simulink library "Linkage_Decoupled_DW"  (R2026a)
settings: Solver=VariableStepAuto
undefined symbols (not defined in the file): Ac, Af, Ar, InitLinkage, Left, Linkage, Visual, X, Y, Z
libraries: sm_lib x48, Suspension_Utilities x27, fl_lib x1, nesl_utility x1
(part 1 of 2)
Description:
  | Component of Simscape Vehicle Templates Library
  | 
  | Copyright 2018-2024 The MathWorks, Inc.
settings Model: Creator=smiller  LastModifiedBy=andrei

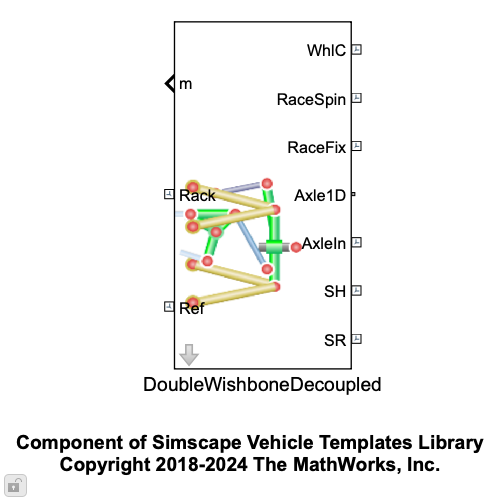
[thumbnail: Simulink's stored preview of the top-level diagram]
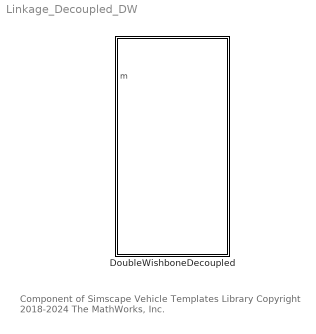
== system Linkage_Decoupled_DW ==
  note: Component of Simscape Vehicle Templates Library
      | Copyright 2018-2024 The MathWorks, Inc.
  DoubleWishboneDecoupled : Subsystem  VariantControl=DWDecoupled  mask(Double-Wishbone Suspension, Decoupled){popup_leftRight=Left, hp_in_f_ua=Linkage.UpperWishbone.sInboardF.Value, hp_in_r_ua=Linkage.UpperWishbone.sInboardR.Value, hp_out_ua=Linkage.UpperWishbone.sOutboard.Value, hp_in_f_la=Linkage.LowerWishbone.sInboardF.Value, hp_in_r_la=Linkage.LowerWishbone.sInboardR.Value, hp_out_la=Linkage.LowerWishbone.sOutboard.Value, hp_pushrod_in=Linkage.Pushrod.sBellcrank.Value, hp_pushrod_out=Linkage.Pushrod.sUpright.Value, hp_bcr_pivot=Linkage.Bellcrank.sPivot.Value, hp_bcr_shock_heaveL=Linkage.Shock.Heave.sLeft.Value, hp_bcr_shock_heaveR=Linkage.Shock.Heave.sRight.Value, hp_bcr_shock_rollL=Linkage.Shock.Roll.sLeft.Value, hp_bcr_shock_rollR=Linkage.Shock.Roll.sRight.Value, hp_upr_cg=Linkage.Upright.sCG.Value, hp_upr_wc=Linkage.Upright.sWheelCentre.Value, hp_in_rod=Linkage.TrackRod.sInboard.Value, hp_upr_rod=Linkage.TrackRod.sOutboard.Value, clr_hp=Visual.hp.clr, opc_hp=Visual.hp.opc, size_hp=Visual.hp.rad, Upper_Arm_to_Subframe=Linkage.Upper_Arm_to_Subframe, ua_mass=Linkage.UpperWishbone.m.Value, clr_ua=Visual.UpperArm.clr, opc_ua=Visual.part.opc, radius_ua=Visual.UpperArm.rad, Lower_Arm_to_Subframe=Linkage.Lower_Arm_to_Subframe, la_mass=Linkage.LowerWishbone.m.Value, clr_la=Visual.LowerArm.clr, opc_la=Visual.part.opc, radius_la=Visual.LowerArm.rad, upr_mass=Linkage.Upright.m.Value, atoe=Linkage.Upright.aToe.Value, acamber=Linkage.Upright.aCamber.Value, axle_len=Linkage.Upright.xAxle.Value, axle_whlc_to_bearing=Linkage.Upright.xWCtoBearing.Value, axle_mass=Linkage.Upright.mAxle.Value, clr_conn_upr=Visual.hp.clr, opc_conn_upr=Visual.hp.opc, size_conn_upr=Visual.hp.rad, clr_upr=Visual.Upright.clr, opc_upr=Visual.part.opc, radius_upr=Visual.Upright.rad, clr_axle=Visual.Axle.clr, opc_axle=Visual.part.opc, radius_axle=Visual.Axle.rad, rod_mass=Linkage.TrackRod.m.Value, clr_conn_rod=Visual.hp.clr, opc_conn_rod=Visual.hp.opc, size_conn_rod=Visual.hp.rad, clr_rod=Visual.TrackRod.clr, opc_rod=Visual.part.opc, radius_rod=Visual.TrackRod.rad, bcr_mass=Linkage.Bellcrank.m.Value, clr_bcr=Visual.Bellcrank.clr, opc_bcr=Visual.part.opc, radius_bcr=Visual.Bellcrank.rad, push_mass=Linkage.Pushrod.m.Value, clr_conn_push=Visual.hp.clr, opc_conn_push=Visual.hp.opc, size_conn_push=Visual.hp.rad, clr_push=Visual.Pushrod.clr, opc_push=Visual.part.opc, radius_push=Visual.Pushrod.rad, whl_init_spd_lr=InitLinkage.nWheel.Value}
      mask prompts: popup_leftRight "Left/Right"; hp_in_f_ua "Upper Arm Front [xyz] (m)"; hp_in_r_ua "Upper Arm Rear [xyz] (m)"; hp_out_ua "Upper Arm Outboard [xyz] (m)"; hp_in_f_la "Lower Arm Front [xyz] (m)"; hp_in_r_la "Lower Arm Rear [xyz] (m)"; hp_out_la "Lower Arm Outboard [xyz] (m)"; hp_pushrod_in "Pushrod Bellcrank [xyz] (m)"; hp_pushrod_out "Pushrod Upright [xyz] (m)"; hp_bcr_pivot "Bellcrank Pivot [xyz] (m)"; hp_bcr_shock_heaveL "Bellcrank Shock Heave Left [xyz] (m)"; hp_bcr_shock_heaveR "Bellcrank Shock Heave Right [xyz] (m)"; hp_bcr_shock_rollL "Bellcrank Shock Roll Left [xyz] (m)"; hp_bcr_shock_rollR "Bellcrank Shock Roll Right [xyz] (m)"; hp_upr_cg "Upright CG [xyz] (m)"; hp_upr_wc "Wheel Center [xyz] (m)"; hp_in_rod "Track Rod Inboard [xyz] (m)"; hp_upr_rod "Track Rod Outboard [xyz] (m)"; Upper_Arm_to_Subframe "Subframe Connection"; ua_mass "Mass (kg)"; clr_ua "Color [RGB]"; opc_ua "Opacity (0-1)"; radius_ua "Radius (m)"; Lower_Arm_to_Subframe "Subframe Connection"; la_mass "Mass (kg)"; clr_la "Color [RGB]"; opc_la "Opacity (0-1)"; radius_la "Radius (m)"; upr_mass "Mass (kg)"; atoe "Toe Angle (deg)"; acamber "Camber Angle (deg)"; axle_len "Axle Length (m)"; axle_whlc_to_bearing "Distance Wheel Ctr to Bearing (m)"; axle_mass "Axle Mass (kg)"; rod_mass "Mass (kg)"; bcr_mass "Mass (kg)"; push_mass "Mass (kg)"; whl_init_spd_lr "Initial Wheel Speed (rad/s)"
      mask help: This models a double-wishbone, decoupled suspension for steered configurations. Mechanical connections via a bellcrank permit this design to decouple stiffness and damping for body roll and heave.
      mask init:
      | if(popup_leftRight == 1)
      |     rhs_susp = 1;
      |     %whlind = 1;
      |     whl_init_spd = whl_init_spd_lr(1);
      |     hp_bcr_shock_heave = hp_bcr_shock_heaveL;
      |     hp_bcr_shock_roll = hp_bcr_shock_rollL;
      | elseif(popup_leftRight == 2)
      |     rhs_susp = -1;
      |     %whlind = 2;
      | 	whl_init_spd = whl_init_spd_lr(2);
      |     hp_bcr_shock_heave = hp_bcr_shock_heaveR;
      |     hp_bcr_shock_roll = hp_bcr_shock_rollR;
      | end
      mask Help: web('sm_car_doc_susp_double_wishbone.html')
      mask TypeOptions popup_leftRight: Hardpoints/popup_leftRight | Lower Arm/popup_leftRight | Upper Arm/popup_leftRight | Upright/popup_leftRight | Track Rod/popup_leftRight | Bellcrank/popup_leftRight | HP Bellcrank/popup_leftRight | Pushrod/popup_leftRight
      mask TypeOptions hp_in_f_ua: Upper Arm/hp_in_f | Hardpoints/hp_in_f_ua
      mask TypeOptions hp_in_r_ua: Upper Arm/hp_in_r | Hardpoints/hp_in_r_ua
      mask TypeOptions hp_out_ua: Upper Arm/hp_out | Upright/hp_ua_out
      mask TypeOptions hp_in_f_la: Hardpoints/hp_in_f_la | Lower Arm/hp_in_f
      mask TypeOptions hp_in_r_la: Hardpoints/hp_in_r_la | Lower Arm/hp_in_r
      mask TypeOptions hp_out_la: Upright/hp_la_out | Lower Arm/hp_out
      mask TypeOptions hp_pushrod_in: Pushrod/hp_in | Bellcrank/hp_pushrod | HP Bellcrank/hp_pushrod_in
      mask TypeOptions hp_pushrod_out: Pushrod/hp_out | Upright/hp_pushrod
      mask TypeOptions hp_bcr_pivot: Bellcrank/hp_bcr_pivot | HP Bellcrank/hp_bcr_pivot | Hardpoints/hp_bellcrank
      mask TypeOptions hp_upr_cg: Upright/hp_upr_cg
      mask TypeOptions hp_upr_wc: Upright/hp_upr_wc
      mask TypeOptions hp_in_rod: Track Rod/hp_in
      mask TypeOptions hp_upr_rod: Track Rod/hp_out | Upright/hp_upr_rod
      mask TypeOptions clr_hp: Hardpoints/clr_hp
      mask TypeOptions opc_hp: Hardpoints/opc_hp
      mask TypeOptions size_hp: Hardpoints/size_hp
      mask TypeOptions ua_mass: Upper Arm/ua_mass
      mask TypeOptions clr_ua: Upper Arm/clr_ua
      mask TypeOptions opc_ua: Upper Arm/opc_ua
      mask TypeOptions radius_ua: Upper Arm/radius_ua
      mask TypeOptions la_mass: Lower Arm/arm_mass
      mask TypeOptions clr_la: Lower Arm/clr_arm
      mask TypeOptions opc_la: Lower Arm/opc_arm
      mask TypeOptions radius_la: Lower Arm/radius_arm
      mask TypeOptions upr_mass: Upright/upr_mass
      mask TypeOptions atoe: Upright/atoe
      mask TypeOptions acamber: Upright/acamber
      mask TypeOptions axle_len: Upright/axle_len
      mask TypeOptions axle_whlc_to_bearing: Upright/axle_whlc_to_bearing
      mask TypeOptions axle_mass: Upright/axle_mass
      mask TypeOptions clr_conn_upr: Upright/clr_conn_upr
      mask TypeOptions opc_conn_upr: Upright/opc_conn_upr
      mask TypeOptions size_conn_upr: Upright/size_conn_upr
      mask TypeOptions clr_upr: Upright/clr_upr
      mask TypeOptions opc_upr: Upright/opc_upr
      mask TypeOptions radius_upr: Upright/radius_upr
      mask TypeOptions clr_axle: Upright/clr_axle
      mask TypeOptions opc_axle: Upright/opc_axle
      mask TypeOptions radius_axle: Upright/radius_axle
      mask TypeOptions rod_mass: Track Rod/rod_mass
      mask TypeOptions clr_conn_rod: Track Rod/clr_conn_rod
      mask TypeOptions opc_conn_rod: Track Rod/opc_conn_rod
      mask TypeOptions size_conn_rod: Track Rod/size_conn_rod
      mask TypeOptions clr_rod: Track Rod/clr_rod
      mask TypeOptions opc_rod: Track Rod/opc_rod
      mask TypeOptions radius_rod: Track Rod/radius_rod
      mask TypeOptions bcr_mass: Bellcrank/bcr_mass
      mask TypeOptions clr_bcr: Bellcrank/clr_bcr
      mask TypeOptions opc_bcr: Bellcrank/opc_bcr
      mask TypeOptions radius_bcr: Bellcrank/radius_bcr
      mask TypeOptions push_mass: Pushrod/rod_mass
      mask TypeOptions clr_conn_push: Pushrod/clr_conn_rod
      mask TypeOptions opc_conn_push: Pushrod/opc_conn_rod
      mask TypeOptions size_conn_push: Pushrod/size_conn_rod
      mask TypeOptions clr_push: Pushrod/clr_rod
      mask TypeOptions opc_push: Pushrod/opc_rod
      mask TypeOptions radius_push: Pushrod/radius_rod
      mask DialogControl cont_hp Prompt: Hardpoints
      mask DialogControl cont_vis_hp Prompt: Visualization
      mask DialogControl text_clr_hp Prompt: Color [RGB]
      mask DialogControl text_opc_hp Prompt: Opac. (0-1)
      mask DialogControl text_size_hp Prompt: Size (m)
      mask DialogControl text_hp Prompt: Hardpoints
      mask DialogControl cont_ua Prompt: UA
      mask DialogControl cont_vis_ua Prompt: Visualization
      mask DialogControl cont_la Prompt: LA
      mask DialogControl cont_vis_la Prompt: Visualization
      mask DialogControl cont_upright Prompt: Upright
      mask DialogControl grp_upright Prompt: Upright
      mask DialogControl grp_upright_axle Prompt: Axle
      mask DialogControl cont_vis_upr Prompt: Visualization
      mask DialogControl text_clr_upr Prompt: Color [RGB]
      mask DialogControl text_opc_upr Prompt: Opac. (0-1)
      mask DialogControl text_size_upr Prompt: Size (m)
      mask DialogControl text_conn_upr Prompt: Connections
      mask DialogControl text_upright Prompt: Upright
      mask DialogControl text_axle Prompt: Axle
      mask DialogControl cont_steer Prompt: Steer
      mask DialogControl grp_rod Prompt: Rod
      mask DialogControl cont_vis_rod Prompt: Visualization
      mask DialogControl text_clr_rod Prompt: Color [RGB]
      mask DialogControl text_opc_rod Prompt: Opac. (0-1)
      mask DialogControl text_size_rod Prompt: Size (m)
      mask DialogControl text_conn_rod Prompt: Connections
      mask DialogControl text_rod_rod Prompt: Rod
      mask DialogControl cont_bellcrank Prompt: Bellcrank
      mask DialogControl grp_bellcrank Prompt: Bellcrank
      mask DialogControl cont_vis_bellcrank Prompt: Visualization
      mask DialogControl text_clr_bellcrank Prompt: Color [RGB]
      mask DialogControl text_opc_bellcrank Prompt: Opac. (0-1)
      mask DialogControl text_size_bellcrank Prompt: Size (m)
      mask DialogControl text_bellcrank Prompt: Bellcrank
      mask DialogControl cont_push Prompt: Pushrod
      mask DialogControl cont_vis_pushrod Prompt: Visualization
      mask DialogControl text_clr_push Prompt: Color [RGB]
      mask DialogControl text_opc_push Prompt: Opac. (0-1)
      mask DialogControl text_size_push Prompt: Size (m)
      mask DialogControl text_push Prompt: Connections
      mask DialogControl text_rod Prompt: Rod
      mask DialogControl cont_init Prompt: Initial
      mask Display: image('sm_car_vehicle_linkage_dwdec_IMAGE.png');

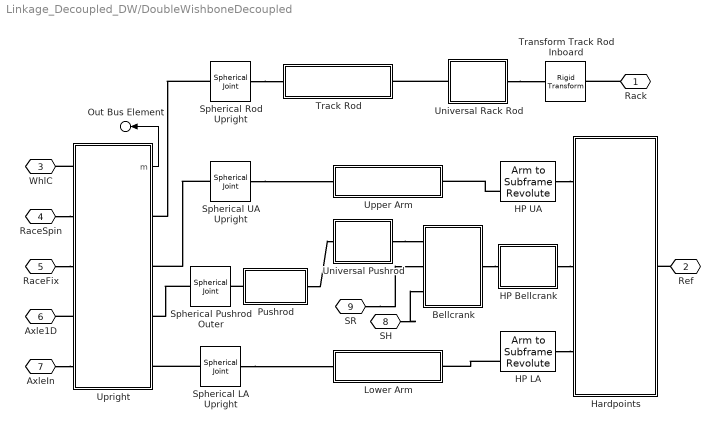
== system Linkage_Decoupled_DW/DoubleWishboneDecoupled ==
  Bellcrank : Subsystem  mask(Bellcrank){popup_leftRight=Left, hp_bcr_pivot=hp_bcr_pivot, hp_bcr_shock_heave=hp_bcr_shock_heave, hp_bcr_shock_roll=hp_bcr_shock_roll, hp_pushrod=hp_pushrod_in, bcr_mass=bcr_mass, clr_bcr=clr_bcr, opc_bcr=opc_bcr, radius_bcr=radius_bcr}
      mask prompts: popup_leftRight "Left/Right"; hp_bcr_pivot "HP Bellcrank Pivot [xyz] (m)"; hp_bcr_shock_heave "HP Bellcrank Shock Heave [xyz] (m)"; hp_bcr_shock_roll "HP Bellcrank Shock Roll [xyz] (m)"; hp_pushrod "HP Bellcrank Pushrod [xyz] (m)"; bcr_mass "Mass (kg)"; clr_bcr "Color [RGB]"; opc_bcr "Opacity (0-1)"; radius_bcr "Radius (m)"
      mask help: Models a bellcrank with one pivot and 3 attachment points. The axis of the pivot is normal to the plane formed by the pivot, connection to the pushrod, and connection to the shock.
      mask init:
      | if(popup_leftRight == 1)
      |     rhs_susp = 1;
      |     %hp_shock_roll = hp_bcr_shock_roll; % Use left value
      | elseif(popup_leftRight == 2)
      |     rhs_susp = -1;
      |     % Code to mirror hardpoint about vehicle xz plane 
      |     % and the plane defined by the bellcrank pivot axis
      |     % and the y axis of the vehicle
      |     % Code not used so that points can be specified independently
      |     % Left here as a reference.
      |     %{
      |     a1 = atan2(hp_pushrod(1)-hp_bcr_pivot(1)   ,hp_pushrod(3)-hp_bcr_pivot(3));
      |     a2 = atan2(hp_bcr_shock_roll(1)-hp_bcr_pivot(1),hp_bcr_shock_roll(3)-hp_bcr_pivot(3));
      |     d_roll2piv = norm(hp_bcr_shock_roll([1 3])-hp_bcr_pivot([1 3]));
      |     d_roll_mirror_axis = d_roll2piv*cos(a2-a1);
      |     mirr_dx = d_roll_mirror_axis*sin(a1);
      |     mirr_dz = d_roll_mirror_axis*cos(a1);
      |     hp_shock_roll = ...
      |         [hp_bcr_shock_roll(1)-2*mirr_dx -hp_bcr_shock_roll(2) hp_bcr_shock_roll(3)-2*mirr_dz];
      |     %}
      | end
      | 
      | rhs_hp = [1 rhs_susp 1];
      mask TypeOptions popup_leftRight: Left | Right
      mask TypeOptions clr_bcr: Arm Pivot Shock Roll/clr_solid | Arm Pivot Push/clr_solid | Arm Pivot Shock Heave/clr_solid | Arm Push Shock/clr_solid
      mask TypeOptions opc_bcr: Arm Pivot Shock Roll/opc_solid | Arm Pivot Push/opc_solid | Arm Pivot Shock Heave/opc_solid | Arm Push Shock/opc_solid
      mask TypeOptions radius_bcr: Arm Pivot Shock Roll/rad_solid | Arm Pivot Push/rad_solid | Arm Pivot Shock Heave/rad_solid | Arm Push Shock/rad_solid
      mask DialogControl cont_ua Prompt: UA
      mask DialogControl cont_vis_ua Prompt: Visualization
      mask Display: image('sm_car_vehicle_linkage_bellcrank_IMAGE.png');
  HP Bellcrank : Subsystem  mask(Revolute Joint 3 Points){popup_leftRight=Left, hp_bcr_pivot=hp_bcr_pivot, hp_pushrod_in=hp_pushrod_in, hp_bcr_shock=hp_bcr_shock_heave}
      mask prompts: popup_leftRight "Left/Right"; hp_bcr_pivot "HP Bellcrank Pivot [xyz] (m)"; hp_pushrod_in "HP Pushrod Inner [xyz] (m)"; hp_bcr_shock "HP Bellcrank Shock Heave [xyz] (m)"
      mask help: Revolute Joint with degree of freedom normal to 3 hardpoints.
      mask init:
      | % Set parameter for mirroring (+y or -y)
      | if(popup_leftRight == 1)
      |     rhs_susp = 1;    
      | elseif(popup_leftRight == 2)
      |     rhs_susp = -1;
      | end
      | 
      | rhs_hp = [1 rhs_susp 1];
      mask TypeOptions popup_leftRight: Left | Right
      mask Display: image('sm_car_variant_revolute.png')
  HP LA : Suspension_Utilities/Arm to Subframe Revolute  VariantControl=Variant1  LabelModeActiveChoice=Bushing_AxRad  popup_leftRight=Left  hp_f=hp_in_f_ua  hp_r=hp_in_r_ua  Connection=Lower_Arm_to_Subframe  VariantLabel=Lower_Arm_to_Subframe.class.Value
      settings: AttributesFormatString=%<ActiveVariant>  SourceProductName=SmCar - Suspension Utilites
  HP UA : Suspension_Utilities/Arm to Subframe Revolute  VariantControl=Variant1  LabelModeActiveChoice=Bushing_AxRad  popup_leftRight=Left  hp_f=hp_in_f_ua  hp_r=hp_in_r_ua  Connection=Upper_Arm_to_Subframe  VariantLabel=Upper_Arm_to_Subframe.class.Value
      settings: AttributesFormatString=%<ActiveVariant>  SourceProductName=SmCar - Suspension Utilites
  Hardpoints : Subsystem  mask{popup_leftRight=Left, hp_in_f_ua=hp_in_f_ua, hp_in_r_ua=hp_in_r_ua, hp_in_f_la=hp_in_f_la, hp_in_r_la=hp_in_r_la, hp_bellcrank=hp_bcr_pivot, clr_hp=clr_hp, opc_hp=opc_hp, size_hp=size_hp}
      mask prompts: popup_leftRight "Left/Right"; hp_in_f_ua "Upper Arm Front [xyz] (m)"; hp_in_r_ua "Upper Arm Rear [xyz] (m)"; hp_in_f_la "Lower Arm Front [xyz] (m)"; hp_in_r_la "Lower Arm Rear [xyz] (m)"; hp_bellcrank "Bellcrank Pivot [xyz] (m)"
      mask init:
      | % Set parameter for mirroring (+y or -y)
      | if(popup_leftRight == 1)
      |     rhs_susp = 1;    
      | elseif(popup_leftRight == 2)
      |     rhs_susp = -1;
      | end
      | 
      | rhs_hp = [1 rhs_susp 1];
      mask TypeOptions popup_leftRight: Left | Right
      mask TypeOptions clr_hp: Subsystem/Vis HP LAf/GraphicDiffuseColor | Vis HP LAr/GraphicDiffuseColor | Vis HP Bellcrank/GraphicDiffuseColor | Vis HP UAf/GraphicDiffuseColor | Vis HP UAr/GraphicDiffuseColor
      mask TypeOptions opc_hp: Subsystem/Vis HP LAf/GraphicOpacity | Vis HP LAr/GraphicOpacity | Vis HP Bellcrank/GraphicOpacity | Vis HP UAf/GraphicOpacity | Vis HP UAr/GraphicOpacity
      mask DialogControl cont_hp Prompt: Hardpoints
      mask DialogControl cont_vis_hp Prompt: Visualization
      mask DialogControl text_clr_hp Prompt: Color [RGB]
      mask DialogControl text_opc_hp Prompt: Opac. (0-1)
      mask DialogControl text_size_hp Prompt: Size (m)
      mask DialogControl text_hp Prompt: Hardpoints
      mask Display: image('sm_car_vehicle_linkage_dw_hp_IMAGE.png');
  Lower Arm : Subsystem  mask{popup_leftRight=Left, hp_in_f=hp_in_f_la, hp_in_r=hp_in_r_la, hp_out=hp_out_la, arm_mass=la_mass, clr_arm=clr_la, opc_arm=opc_la, radius_arm=radius_la}
      mask prompts: popup_leftRight "Left/Right"; hp_in_f "Inboard Front [xyz] (m)"; hp_in_r "Inboard Rear [xyz] (m)"; hp_out "Outboard [xyz] (m)"; arm_mass "Mass (kg)"; clr_arm "Color [RGB]"; opc_arm "Opacity (0-1)"; radius_arm "Radius (m)"
      mask init:
      | if(popup_leftRight == 1)
      |     rhs_susp = 1;
      | elseif(popup_leftRight == 2)
      |     rhs_susp = -1;
      | end
      | 
      | rhs_hp = [1 rhs_susp 1];
      mask TypeOptions popup_leftRight: Left | Right
      mask TypeOptions clr_arm: Arm F/clr_solid | Arm R/clr_solid
      mask TypeOptions opc_arm: Arm F/opc_solid | Arm R/opc_solid
      mask TypeOptions radius_arm: Arm F/rad_solid | Arm R/rad_solid
      mask DialogControl cont_ua Prompt: LA
      mask DialogControl cont_vis_arm Prompt: Visualization
      mask Display: image('sm_car_vehicle_linkage_dw_ua_IMAGE.png');
  Pushrod : Subsystem  VariantControl=Steer  mask{popup_leftRight=Left, hp_in=hp_pushrod_in, hp_out=hp_pushrod_out, rod_mass=push_mass, clr_conn_rod=clr_conn_push, opc_conn_rod=opc_conn_push, size_conn_rod=size_conn_push, clr_rod=clr_push, opc_rod=opc_push, radius_rod=radius_push}
      mask prompts: popup_leftRight "Left/Right"; hp_in "Inboard [xyz] (m)"; hp_out "Outboard [xyz] (m)"; rod_mass "Mass (kg)"
      mask init:
      | if(popup_leftRight == 1)
      |     rhs_rod = 1;
      | elseif(popup_leftRight == 2)
      |     rhs_rod = -1;
      | end
      mask TypeOptions popup_leftRight: Left | Right
      mask TypeOptions rod_mass: Arm/Mass
      mask TypeOptions clr_conn_rod:
      | Vis
      | Upright
      | Steer/GraphicDiffuseColor | Vis
      | Rack
      | Rod/GraphicDiffuseColor
      mask TypeOptions opc_conn_rod:
      | Vis
      | Upright
      | Steer/GraphicOpacity | Vis
      | Rack
      | Rod/GraphicOpacity
      mask TypeOptions clr_rod: Arm/clr_solid
      mask TypeOptions opc_rod: Arm/opc_solid
      mask TypeOptions radius_rod: Arm/rad_solid
      mask DialogControl cont_rod Prompt: Rod
      mask DialogControl grp_rod Prompt: Rod
      mask DialogControl cont_vis_rod Prompt: Visualization
      mask DialogControl text_clr_rod Prompt: Color [RGB]
      mask DialogControl text_opc_rod Prompt: Opacity (0-1)
      mask DialogControl text_size_rod Prompt: Radius (m)
      mask DialogControl text_conn_rod Prompt: Connections
      mask DialogControl text_rod_rod Prompt: Rod
      mask Display: image('sm_car_vehicle_linkage_link_IMAGE.png');
  Spherical LA Upright : sm_lib/Joints/Spherical Joint  JointMode=Normal  CompositeWrenchDir=FollowerOnBase  CompositeWrenchFrame=BaseFrame  SenseConstraintForce=off  SenseConstraintTorque=off  SenseTotalForce=off  SenseTotalTorque=off  PositionTargetSpecify=off  PositionTargetPriority=High  PositionTargetRotationMethod=None  PositionTargetFollAlignAxisA=+X  PositionTargetBaseAlignAxisA=+Y  PositionTargetFollAlignAxisB=+Y  PositionTargetBaseAlignAxisB=+Z  PositionTargetRotationStandardAxis=+Z  PositionTargetRotationAngle=0.0  PositionTargetRotationAngleUnits=deg  PositionTargetRotationArbitraryAxis=[0 0 1]  PositionTargetRotationSequenceAxes=FollowerAxes  PositionTargetRotationSequence=XYX  PositionTargetRotationSequenceAngles=[0 0 0]  PositionTargetRotationSequenceAnglesUnits=deg  PositionTargetRotationMatrix=[1 0 0; 0 1 0; 0 0 1]  PositionTargetQuaternion=[1 0 0 0]  VelocityTargetSpecify=off  VelocityTargetPriority=High  VelocityTargetValue=[0 0 0]  VelocityTargetValueUnits=deg/s  VelocityTargetInFollowerFrame=on  EqPosRotationMethod=None  EqPosFollAlignAxisA=+X  EqPosBaseAlignAxisA=+Y  EqPosFollAlignAxisB=+Y  EqPosBaseAlignAxisB=+Z  EqPosRotationStandardAxis=+Z  EqPosRotationAngle=0.0  EqPosRotationAngleUnits=deg  EqPosRotationArbitraryAxis=[0 0 1]  EqPosRotationSequenceAxes=FollowerAxes  EqPosRotationSequence=XYX  EqPosRotationSequenceAngles=[0 0 0]  EqPosRotationSequenceAnglesUnits=deg  EqPosRotationMatrix=[1 0 0; 0 1 0; 0 0 1]  EqPosQuaternion=[1 0 0 0]  SpringStiffness=0  SpringStiffnessUnits=N*m/deg  DampingCoefficient=0  DampingCoefficientUnits=N*m/(deg/s)  LowerLimitSpecify=off  LowerLimitBound=15  LowerLimitBoundUnits=deg  LowerLimitStiffness=1e4  LowerLimitStiffnessUnits=N*m/deg  LowerLimitDamping=10  LowerLimitDampingUnits=N*m/(deg/s)  LowerLimitTransitionRegionWidth=0.1  LowerLimitTransitionRegionWidthUnits=deg  UpperLimitSpecify=off  UpperLimitBound=45  UpperLimitBoundUnits=deg  UpperLimitStiffness=1e4  UpperLimitStiffnessUnits=N*m/deg  UpperLimitDamping=10  UpperLimitDampingUnits=N*m/(deg/s)  UpperLimitTransitionRegionWidth=0.1  UpperLimitTransitionRegionWidthUnits=deg  TorqueActuationMode=NoTorque  ActuateTorqueX=off  ActuateTorqueY=off  ActuateTorqueZ=off  ActuateTorque=off  ActuationFrame=BaseFrame  SensePosition=off  SenseVelocityX=off  SenseVelocityY=off  SenseVelocityZ=off  SenseVelocity=off  SenseAccelerationX=off  SenseAccelerationY=off  SenseAccelerationZ=off  SenseAcceleration=off  SenseLowerLimitTorqueMag=off  SenseUpperLimitTorqueMag=off  SensingFrame=BaseFrame
  Spherical Pushrod Outer : sm_lib/Joints/Spherical Joint  JointMode=Normal  CompositeWrenchDir=FollowerOnBase  CompositeWrenchFrame=BaseFrame  SenseConstraintForce=off  SenseConstraintTorque=off  SenseTotalForce=off  SenseTotalTorque=off  PositionTargetSpecify=on  PositionTargetPriority=Low  PositionTargetRotationMethod=AlignedAxes  PositionTargetFollAlignAxisA=+X  PositionTargetBaseAlignAxisA=+X  PositionTargetFollAlignAxisB=+Y  PositionTargetBaseAlignAxisB=+Y  PositionTargetRotationStandardAxis=+Z  PositionTargetRotationAngle=0.0  PositionTargetRotationAngleUnits=deg  PositionTargetRotationArbitraryAxis=[0 0 1]  PositionTargetRotationSequenceAxes=FollowerAxes  PositionTargetRotationSequence=XYX  PositionTargetRotationSequenceAngles=[0 0 0]  PositionTargetRotationSequenceAnglesUnits=deg  PositionTargetRotationMatrix=[1 0 0; 0 1 0; 0 0 1]  PositionTargetQuaternion=[1 0 0 0]  VelocityTargetSpecify=off  VelocityTargetPriority=High  VelocityTargetValue=[0 0 0]  VelocityTargetValueUnits=deg/s  VelocityTargetInFollowerFrame=on  EqPosRotationMethod=None  EqPosFollAlignAxisA=+X  EqPosBaseAlignAxisA=+Y  EqPosFollAlignAxisB=+Y  EqPosBaseAlignAxisB=+Z  EqPosRotationStandardAxis=+Z  EqPosRotationAngle=0.0  EqPosRotationAngleUnits=deg  EqPosRotationArbitraryAxis=[0 0 1]  EqPosRotationSequenceAxes=FollowerAxes  EqPosRotationSequence=XYX  EqPosRotationSequenceAngles=[0 0 0]  EqPosRotationSequenceAnglesUnits=deg  EqPosRotationMatrix=[1 0 0; 0 1 0; 0 0 1]  EqPosQuaternion=[1 0 0 0]  SpringStiffness=0  SpringStiffnessUnits=N*m/deg  DampingCoefficient=0  DampingCoefficientUnits=N*m/(deg/s)  LowerLimitSpecify=off  LowerLimitBound=15  LowerLimitBoundUnits=deg  LowerLimitStiffness=1e4  LowerLimitStiffnessUnits=N*m/deg  LowerLimitDamping=10  LowerLimitDampingUnits=N*m/(deg/s)  LowerLimitTransitionRegionWidth=0.1  LowerLimitTransitionRegionWidthUnits=deg  UpperLimitSpecify=off  UpperLimitBound=45  UpperLimitBoundUnits=deg  UpperLimitStiffness=1e4  UpperLimitStiffnessUnits=N*m/deg  UpperLimitDamping=10  UpperLimitDampingUnits=N*m/(deg/s)  UpperLimitTransitionRegionWidth=0.1  UpperLimitTransitionRegionWidthUnits=deg  TorqueActuationMode=NoTorque  ActuateTorqueX=off  ActuateTorqueY=off  ActuateTorqueZ=off  ActuateTorque=off  ActuationFrame=BaseFrame  SensePosition=off  SenseVelocityX=off  SenseVelocityY=off  SenseVelocityZ=off  SenseVelocity=off  SenseAccelerationX=off  SenseAccelerationY=off  SenseAccelerationZ=off  SenseAcceleration=off  SenseLowerLimitTorqueMag=off  SenseUpperLimitTorqueMag=off  SensingFrame=BaseFrame
  Spherical Rod Upright : sm_lib/Joints/Spherical Joint  JointMode=Normal  CompositeWrenchDir=FollowerOnBase  CompositeWrenchFrame=BaseFrame  SenseConstraintForce=off  SenseConstraintTorque=off  SenseTotalForce=off  SenseTotalTorque=off  PositionTargetSpecify=off  PositionTargetPriority=High  PositionTargetRotationMethod=None  PositionTargetFollAlignAxisA=+X  PositionTargetBaseAlignAxisA=+Y  PositionTargetFollAlignAxisB=+Y  PositionTargetBaseAlignAxisB=+Z  PositionTargetRotationStandardAxis=+Z  PositionTargetRotationAngle=0.0  PositionTargetRotationAngleUnits=deg  PositionTargetRotationArbitraryAxis=[0 0 1]  PositionTargetRotationSequenceAxes=FollowerAxes  PositionTargetRotationSequence=XYX  PositionTargetRotationSequenceAngles=[0 0 0]  PositionTargetRotationSequenceAnglesUnits=deg  PositionTargetRotationMatrix=[1 0 0; 0 1 0; 0 0 1]  PositionTargetQuaternion=[1 0 0 0]  VelocityTargetSpecify=off  VelocityTargetPriority=High  VelocityTargetValue=[0 0 0]  VelocityTargetValueUnits=deg/s  VelocityTargetInFollowerFrame=on  EqPosRotationMethod=None  EqPosFollAlignAxisA=+X  EqPosBaseAlignAxisA=+Y  EqPosFollAlignAxisB=+Y  EqPosBaseAlignAxisB=+Z  EqPosRotationStandardAxis=+Z  EqPosRotationAngle=0.0  EqPosRotationAngleUnits=deg  EqPosRotationArbitraryAxis=[0 0 1]  EqPosRotationSequenceAxes=FollowerAxes  EqPosRotationSequence=XYX  EqPosRotationSequenceAngles=[0 0 0]  EqPosRotationSequenceAnglesUnits=deg  EqPosRotationMatrix=[1 0 0; 0 1 0; 0 0 1]  EqPosQuaternion=[1 0 0 0]  SpringStiffness=0  SpringStiffnessUnits=N*m/deg  DampingCoefficient=0  DampingCoefficientUnits=N*m/(deg/s)  LowerLimitSpecify=off  LowerLimitBound=15  LowerLimitBoundUnits=deg  LowerLimitStiffness=1e4  LowerLimitStiffnessUnits=N*m/deg  LowerLimitDamping=10  LowerLimitDampingUnits=N*m/(deg/s)  LowerLimitTransitionRegionWidth=0.1  LowerLimitTransitionRegionWidthUnits=deg  UpperLimitSpecify=off  UpperLimitBound=45  UpperLimitBoundUnits=deg  UpperLimitStiffness=1e4  UpperLimitStiffnessUnits=N*m/deg  UpperLimitDamping=10  UpperLimitDampingUnits=N*m/(deg/s)  UpperLimitTransitionRegionWidth=0.1  UpperLimitTransitionRegionWidthUnits=deg  TorqueActuationMode=NoTorque  ActuateTorqueX=off  ActuateTorqueY=off  ActuateTorqueZ=off  ActuateTorque=off  ActuationFrame=BaseFrame  SensePosition=off  SenseVelocityX=off  SenseVelocityY=off  SenseVelocityZ=off  SenseVelocity=off  SenseAccelerationX=off  SenseAccelerationY=off  SenseAccelerationZ=off  SenseAcceleration=off  SenseLowerLimitTorqueMag=off  SenseUpperLimitTorqueMag=off  SensingFrame=BaseFrame
  Spherical UA Upright : sm_lib/Joints/Spherical Joint  JointMode=Normal  CompositeWrenchDir=FollowerOnBase  CompositeWrenchFrame=BaseFrame  SenseConstraintForce=off  SenseConstraintTorque=off  SenseTotalForce=off  SenseTotalTorque=off  PositionTargetSpecify=on  PositionTargetPriority=High  PositionTargetRotationMethod=StandardAxis  PositionTargetFollAlignAxisA=+X  PositionTargetBaseAlignAxisA=+Y  PositionTargetFollAlignAxisB=+Y  PositionTargetBaseAlignAxisB=+Z  PositionTargetRotationStandardAxis=+Z  PositionTargetRotationAngle=0.0  PositionTargetRotationAngleUnits=deg  PositionTargetRotationArbitraryAxis=[0 0 1]  PositionTargetRotationSequenceAxes=FollowerAxes  PositionTargetRotationSequence=XYX  PositionTargetRotationSequenceAngles=[0 0 0]  PositionTargetRotationSequenceAnglesUnits=deg  PositionTargetRotationMatrix=[1 0 0; 0 1 0; 0 0 1]  PositionTargetQuaternion=[1 0 0 0]  VelocityTargetSpecify=off  VelocityTargetPriority=High  VelocityTargetValue=[0 0 0]  VelocityTargetValueUnits=deg/s  VelocityTargetInFollowerFrame=on  EqPosRotationMethod=None  EqPosFollAlignAxisA=+X  EqPosBaseAlignAxisA=+Y  EqPosFollAlignAxisB=+Y  EqPosBaseAlignAxisB=+Z  EqPosRotationStandardAxis=+Z  EqPosRotationAngle=0.0  EqPosRotationAngleUnits=deg  EqPosRotationArbitraryAxis=[0 0 1]  EqPosRotationSequenceAxes=FollowerAxes  EqPosRotationSequence=XYX  EqPosRotationSequenceAngles=[0 0 0]  EqPosRotationSequenceAnglesUnits=deg  EqPosRotationMatrix=[1 0 0; 0 1 0; 0 0 1]  EqPosQuaternion=[1 0 0 0]  SpringStiffness=0  SpringStiffnessUnits=N*m/deg  DampingCoefficient=0  DampingCoefficientUnits=N*m/(deg/s)  LowerLimitSpecify=off  LowerLimitBound=15  LowerLimitBoundUnits=deg  LowerLimitStiffness=1e4  LowerLimitStiffnessUnits=N*m/deg  LowerLimitDamping=10  LowerLimitDampingUnits=N*m/(deg/s)  LowerLimitTransitionRegionWidth=0.1  LowerLimitTransitionRegionWidthUnits=deg  UpperLimitSpecify=off  UpperLimitBound=45  UpperLimitBoundUnits=deg  UpperLimitStiffness=1e4  UpperLimitStiffnessUnits=N*m/deg  UpperLimitDamping=10  UpperLimitDampingUnits=N*m/(deg/s)  UpperLimitTransitionRegionWidth=0.1  UpperLimitTransitionRegionWidthUnits=deg  TorqueActuationMode=NoTorque  ActuateTorqueX=off  ActuateTorqueY=off  ActuateTorqueZ=off  ActuateTorque=off  ActuationFrame=BaseFrame  SensePosition=off  SenseVelocityX=off  SenseVelocityY=off  SenseVelocityZ=off  SenseVelocity=off  SenseAccelerationX=off  SenseAccelerationY=off  SenseAccelerationZ=off  SenseAcceleration=off  SenseLowerLimitTorqueMag=off  SenseUpperLimitTorqueMag=off  SensingFrame=BaseFrame
  Track Rod : Subsystem  VariantControl=Steer  mask{popup_leftRight=Left, hp_in=hp_in_rod, hp_out=hp_upr_rod, rod_mass=rod_mass, clr_conn_rod=clr_conn_rod, opc_conn_rod=opc_conn_rod, size_conn_rod=size_conn_rod, clr_rod=clr_rod, opc_rod=opc_rod, radius_rod=radius_rod}
      mask prompts: popup_leftRight "Left/Right"; hp_in "Inboard [xyz] (m)"; hp_out "Outboard [xyz] (m)"; rod_mass "Mass (kg)"; clr_rod "Color [RGB]"; opc_rod "Opacity (0-1)"; radius_rod "Radius (m)"
      mask init:
      | if(popup_leftRight == 1)
      |     rhs_rod = 1;
      | elseif(popup_leftRight == 2)
      |     rhs_rod = -1;
      | end
      mask TypeOptions popup_leftRight: Left | Right
      mask TypeOptions rod_mass: Rod/Mass
      mask TypeOptions clr_conn_rod:
      | Vis
      | Upright
      | Steer/GraphicDiffuseColor | Vis
      | Rack
      | Rod/GraphicDiffuseColor
      mask TypeOptions opc_conn_rod:
      | Vis
      | Upright
      | Steer/GraphicOpacity | Vis
      | Rack
      | Rod/GraphicOpacity
      mask TypeOptions clr_rod: Rod/clr_solid
      mask TypeOptions opc_rod: Rod/opc_solid
      mask TypeOptions radius_rod: Rod/rad_solid
      mask DialogControl cont_rod Prompt: Rod
      mask DialogControl grp_rod Prompt: Rod
      mask DialogControl cont_vis_rod Prompt: Visualization
      mask DialogControl text_clr_rod Prompt: Color [RGB]
      mask DialogControl text_opc_rod Prompt: Opac. (0-1)
      mask DialogControl text_size_rod Prompt: Size (m)
      mask DialogControl text_conn_rod Prompt: Connections
      mask DialogControl text_rod_rod Prompt: Rod
      mask Display: image('sm_car_linkage_trackrod_IMAGE.png');
  Transform Track Rod Inboard : sm_lib/Frames and Transforms/Rigid Transform  RotationMethod=None  FollAlignAxisA=+X  BaseAlignAxisA=+Y  FollAlignAxisB=+Y  BaseAlignAxisB=+Z  RotationStandardAxis=+Z  RotationAngle=0.0  RotationAngleUnits=deg  RotationArbitraryAxis=[0 0 1]  RotationSequenceAxes=FollowerAxes  RotationSequence=XYX  RotationSequenceAngles=[0 0 0]  RotationSequenceAnglesUnits=deg  RotationMatrix=[1 0 0; 0 1 0; 0 0 1]  Quaternion=[1 0 0 0]  TranslationMethod=Cartesian  TranslationCartesianOffset=hp_in_rod.*[1 rhs_susp 1]  TranslationCartesianOffsetUnits=m  TranslationStandardAxis=+Z  TranslationStandardOffset=0  TranslationStandardOffsetUnits=m  TranslationROffset=0  TranslationROffsetUnits=m  TranslationThetaOffset=0  TranslationThetaOffsetUnits=deg  TranslationZOffset=0  TranslationZOffsetUnits=m
  Universal Pushrod : Subsystem
      mask Display: image('sm_car_variant_universal.png');
  Universal Rack Rod : Subsystem
      mask Display: image('sm_car_variant_universal.png');
  Upper Arm : Subsystem  mask{popup_leftRight=Left, hp_in_f=hp_in_f_ua, hp_in_r=hp_in_r_ua, hp_out=hp_out_ua, ua_mass=ua_mass, clr_ua=clr_ua, opc_ua=opc_ua, radius_ua=radius_ua}
      mask prompts: popup_leftRight "Left/Right"; hp_in_f "Inboard Front [xyz] (m)"; hp_in_r "Inboard Rear [xyz] (m)"; hp_out "Outboard [xyz] (m)"; ua_mass "Mass (kg)"; clr_ua "Color [RGB]"; opc_ua "Opacity (0-1)"; radius_ua "Radius (m)"
      mask init:
      | if(popup_leftRight == 1)
      |     rhs_susp = 1;
      | elseif(popup_leftRight == 2)
      |     rhs_susp = -1;
      | end
      | 
      | rhs_hp = [1 rhs_susp 1];
      mask TypeOptions popup_leftRight: Left | Right
      mask TypeOptions clr_ua: Arm F/clr_solid | Arm R/clr_solid
      mask TypeOptions opc_ua: Arm F/opc_solid | Arm R/opc_solid
      mask TypeOptions radius_ua: Arm F/rad_solid | Arm R/rad_solid
      mask DialogControl cont_ua Prompt: UA
      mask DialogControl cont_vis_ua Prompt: Visualization
      mask Display: image('sm_car_vehicle_linkage_dw_ua_IMAGE.png');
  Upright : Subsystem  mask{popup_leftRight=Left, hp_ua_out=hp_out_ua, hp_la_out=hp_out_la, hp_upr_rod=hp_upr_rod, hp_pushrod=hp_pushrod_out, hp_upr_cg=hp_upr_cg, hp_upr_wc=hp_upr_wc, axle_len=axle_len, axle_whlc_to_bearing=axle_whlc_to_bearing, axle_mass=axle_mass, atoe=atoe, acamber=acamber, upr_mass=upr_mass, whl_init_spd_upr=whl_init_spd, clr_conn_upr=clr_conn_upr, opc_conn_upr=opc_conn_upr, size_conn_upr=size_conn_upr, clr_upr=clr_upr, opc_upr=opc_upr, radius_upr=radius_upr, clr_axle=clr_axle, opc_axle=opc_axle, radius_axle=radius_axle}
      mask prompts: popup_leftRight "Left/Right"; hp_ua_out "Upper Arm Outboard [xyz] (m)"; hp_la_out "Lower Arm Outboard [xyz] (m)"; hp_upr_rod "Track Rod Outboard [xyz] (m)"; hp_pushrod "Pushrod Outboard [xyz] (m)"; hp_upr_cg "Center of Mass [xyz] (m)"; hp_upr_wc "Wheel Center [xyz] (m)"; axle_len "Axle Length (m)"; axle_whlc_to_bearing "Distance Wheel Ctr to Bearing (m)"; axle_mass "Axle Mass (kg)"; atoe "Toe Angle (deg)"; acamber "Camber Angle (deg)"; upr_mass "Upright Mass (kg)"; whl_init_spd_upr "Initial Wheel Speed (rad/s)"
      mask init:
      | % Set parameter for mirroring (+y or -y)
      | if(popup_leftRight == 1)
      |     rhs_upr = 1;
      | elseif(popup_leftRight == 2)
      |     rhs_upr = -1;
      | end
      | rhs_hp = [1 rhs_upr 1];
      | 
      | % Additional hardpoint at center of upright
      | % Used as attachment points for axle and steering arm
      | hp_upr_ctr = (hp_ua_out+hp_la_out)/2;
      mask TypeOptions popup_leftRight: Left | Right
      mask TypeOptions axle_mass: Axle/Mass
      mask TypeOptions upr_mass:
      | Inertia
      | CG/Mass
      mask TypeOptions whl_init_spd_upr: Revolute/whl_init_spd_jnt
      mask TypeOptions clr_conn_upr:
      | Vis Upright LA/GraphicDiffuseColor | Vis Upright UA/GraphicDiffuseColor | Vis Wheel
      | Center/GraphicDiffuseColor
      mask TypeOptions opc_conn_upr:
      | Vis Upright LA/GraphicOpacity | Vis Upright UA/GraphicOpacity | Vis Wheel
      | Center/GraphicOpacity
      mask TypeOptions clr_upr:
      | Upright/clr_solid | Steering Arm/clr_solid | Bearing
      | Carrier/GraphicDiffuseColor | Pushrod Conn/clr_solid
      mask TypeOptions opc_upr: Upright/opc_solid | Steering Arm/opc_solid | Pushrod Conn/opc_solid
      mask TypeOptions radius_upr: Upright/rad_solid | Steering Arm/rad_solid | Pushrod Conn/rad_solid
      mask TypeOptions clr_axle: Axle/GraphicDiffuseColor
      mask TypeOptions opc_axle: Axle/GraphicOpacity
      mask TypeOptions radius_axle: Axle/CylinderRadius
      mask DialogControl cont_upright Prompt: Upright
      mask DialogControl grp_init Prompt: Initialization
      mask DialogControl cont_vis_upr Prompt: Visualization
      mask DialogControl text_clr_upr Prompt: Color [RGB]
      mask DialogControl text_opc_upr Prompt: Opac. (0-1)
      mask DialogControl text_size_upr Prompt: Size (m)
      mask DialogControl text_conn_upr Prompt: Connections
      mask DialogControl text_upright Prompt: Upright
      mask DialogControl text_stub_axle Prompt: Axle
      mask Display: image('sm_car_vehicle_linkage_dw_upr_IMAGE.png');
  Rack : PMIOPort  Side=Right
  Ref : PMIOPort  Port=2  Side=Right
  WhlC : PMIOPort  Port=3  Side=Left
  RaceSpin : PMIOPort  Port=4  Side=Left
  RaceFix : PMIOPort  Port=5  Side=Left
  Axle1D : PMIOPort  Port=6  Side=Left
  AxleIn : PMIOPort  Port=7  Side=Left
  SH : PMIOPort  Port=8  Side=Left
  SR : PMIOPort  Port=9  Side=Left
  Out Bus Element : Outport  VectorParamsAs1DForOutWhenUnconnected=off  PortName=m  Element=Upright
  wires:
  Upright/1(m) -> Out Bus Element/1
  connections:
  Pushrod/RConn1 -- Universal Pushrod/LConn1
  Pushrod/LConn1 -- Spherical Pushrod Outer/LConn1
  SH/RConn1 -- Bellcrank/LConn3
  SR/RConn1 -- Bellcrank/LConn2
  Spherical Pushrod Outer/RConn1 -- Upright/RConn3
  Universal Pushrod/RConn1 -- Bellcrank/LConn1
  Universal Rack Rod/RConn1 -- Transform Track Rod Inboard/RConn1
  Universal Rack Rod/LConn1 -- Track Rod/RConn1
  Spherical Rod Upright/LConn1 -- Track Rod/LConn1
  Spherical UA Upright/RConn1 -- Upright/RConn2
  Spherical LA Upright/LConn1 -- Lower Arm/LConn1
  HP LA/RConn1 -- Lower Arm/RConn1
  Spherical UA Upright/LConn1 -- Upper Arm/LConn1
  Spherical LA Upright/RConn1 -- Upright/RConn4
  HP LA/LConn1 -- Hardpoints/LConn3
  HP UA/RConn1 -- Upper Arm/RConn1
  Upright/LConn4 -- Axle1D/RConn1
  Rack/RConn1 -- Transform Track Rod Inboard/LConn1
  Spherical Rod Upright/RConn1 -- Upright/RConn1
  HP UA/LConn1 -- Hardpoints/LConn1
  Ref/RConn1 -- Hardpoints/RConn1
  HP Bellcrank/LConn1 -- Hardpoints/LConn2
  Upright/LConn1 -- WhlC/RConn1
  Bellcrank/RConn1 -- HP Bellcrank/RConn1
  RaceSpin/RConn1 -- Upright/LConn2
  RaceFix/RConn1 -- Upright/LConn3
  AxleIn/RConn1 -- Upright/LConn5

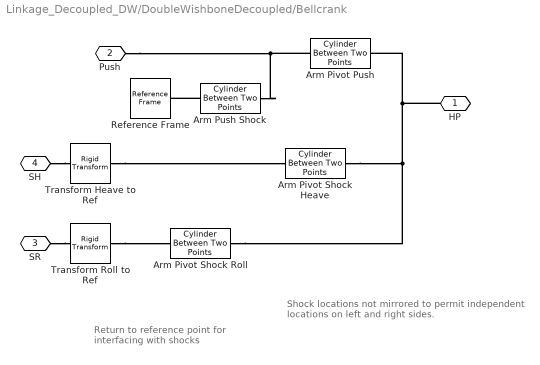
== system Linkage_Decoupled_DW/DoubleWishboneDecoupled/Bellcrank ==
  note: Return to reference point for interfacing with shocks
  note: Shock locations not mirrored to permit independent locations on left and right sides.
  Arm Pivot Push : Suspension_Utilities/Cylinder Between Two Points  hp_b=hp_bcr_pivot.*rhs_hp  hp_f=hp_pushrod.*rhs_hp  Mass=bcr_mass/3  clr_solid=clr_bcr  opc_solid=opc_bcr  rad_solid=radius_bcr
      settings: SourceProductName=SmCar - Suspension Utilites
  Arm Pivot Shock Heave : Suspension_Utilities/Cylinder Between Two Points  hp_b=hp_bcr_pivot.*rhs_hp  hp_f=hp_bcr_shock_heave  Mass=bcr_mass/3  clr_solid=clr_bcr  opc_solid=opc_bcr  rad_solid=radius_bcr
      settings: SourceProductName=SmCar - Suspension Utilites
  Arm Pivot Shock Roll : Suspension_Utilities/Cylinder Between Two Points  hp_b=hp_bcr_pivot.*rhs_hp  hp_f=hp_bcr_shock_roll  Mass=bcr_mass*0.001  clr_solid=clr_bcr  opc_solid=opc_bcr  rad_solid=radius_bcr
      settings: SourceProductName=SmCar - Suspension Utilites
  Arm Push Shock : Suspension_Utilities/Cylinder Between Two Points  hp_b=hp_pushrod.*rhs_hp  hp_f=hp_bcr_shock_heave  Mass=bcr_mass/3  clr_solid=clr_bcr  opc_solid=opc_bcr  rad_solid=radius_bcr
      settings: SourceProductName=SmCar - Suspension Utilites
  Reference Frame : sm_lib/Frames and Transforms/Reference Frame
  Transform Heave to Ref : sm_lib/Frames and Transforms/Rigid Transform  RotationMethod=None  FollAlignAxisA=+X  BaseAlignAxisA=+Y  FollAlignAxisB=+Y  BaseAlignAxisB=+Z  RotationStandardAxis=+Z  RotationAngle=0.0  RotationAngleUnits=deg  RotationArbitraryAxis=[0 0 1]  RotationSequenceAxes=FollowerAxes  RotationSequence=XYX  RotationSequenceAngles=[0 0 0]  RotationSequenceAnglesUnits=deg  RotationMatrix=[1 0 0; 0 1 0; 0 0 1]  Quaternion=[1 0 0 0]  TranslationMethod=Cartesian  TranslationCartesianOffset=hp_bcr_shock_heave  TranslationCartesianOffsetUnits=m  TranslationStandardAxis=+Z  TranslationStandardOffset=0  TranslationStandardOffsetUnits=m  TranslationROffset=0  TranslationROffsetUnits=m  TranslationThetaOffset=0  TranslationThetaOffsetUnits=deg  TranslationZOffset=0  TranslationZOffsetUnits=m
  Transform Roll to Ref : sm_lib/Frames and Transforms/Rigid Transform  RotationMethod=None  FollAlignAxisA=+X  BaseAlignAxisA=+Y  FollAlignAxisB=+Y  BaseAlignAxisB=+Z  RotationStandardAxis=+Z  RotationAngle=0.0  RotationAngleUnits=deg  RotationArbitraryAxis=[0 0 1]  RotationSequenceAxes=FollowerAxes  RotationSequence=XYX  RotationSequenceAngles=[0 0 0]  RotationSequenceAnglesUnits=deg  RotationMatrix=[1 0 0; 0 1 0; 0 0 1]  Quaternion=[1 0 0 0]  TranslationMethod=Cartesian  TranslationCartesianOffset=hp_bcr_shock_roll  TranslationCartesianOffsetUnits=m  TranslationStandardAxis=+Z  TranslationStandardOffset=0  TranslationStandardOffsetUnits=m  TranslationROffset=0  TranslationROffsetUnits=m  TranslationThetaOffset=0  TranslationThetaOffsetUnits=deg  TranslationZOffset=0  TranslationZOffsetUnits=m
  HP : PMIOPort  Side=Right
  Push : PMIOPort  Port=2  Side=Left
  SR : PMIOPort  Port=3  Side=Left
  SH : PMIOPort  Port=4  Side=Left
  connections:
  SR/RConn1 -- Transform Roll to Ref/LConn1
  Arm Push Shock/LConn1 -- Arm Pivot Push/RConn1 -- Push/RConn1
  Arm Pivot Shock Heave/LConn1 -- Arm Pivot Shock Roll/LConn1 -- Arm Pivot Push/LConn1 -- HP/RConn1
  SH/RConn1 -- Transform Heave to Ref/LConn1
  Arm Push Shock/RConn1 -- Reference Frame/RConn1
  Transform Roll to Ref/RConn1 -- Arm Pivot Shock Roll/RConn1
  Transform Heave to Ref/RConn1 -- Arm Pivot Shock Heave/RConn1

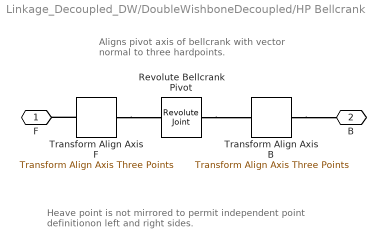
== system Linkage_Decoupled_DW/DoubleWishboneDecoupled/HP Bellcrank ==
  note: Aligns pivot axis of bellcrank with vector normal to three hardpoints.
  note: Heave point is not mirrored to permit independent point definitionon left and right sides.
  Revolute Bellcrank Pivot : sm_lib/Joints/Revolute Joint  JointMode=Normal  CompositeWrenchDir=FollowerOnBase  CompositeWrenchFrame=BaseFrame  SenseConstraintForce=off  SenseConstraintTorque=off  SenseTotalForce=off  SenseTotalTorque=off  PositionTargetSpecify=off  PositionTargetPriority=Low  PositionTargetValue=0  PositionTargetValueUnits=deg  VelocityTargetSpecify=off  VelocityTargetPriority=High  VelocityTargetValue=0  VelocityTargetValueUnits=deg/s  EquilibriumPosition=0  EquilibriumPositionUnits=deg  SpringStiffness=0  SpringStiffnessUnits=N*m/deg  DampingCoefficient=0  DampingCoefficientUnits=N*m/(deg/s)  LowerLimitSpecify=off  LowerLimitBound=-90  LowerLimitBoundUnits=deg  LowerLimitStiffness=1e4  LowerLimitStiffnessUnits=N*m/deg  LowerLimitDamping=10  LowerLimitDampingUnits=N*m/(deg/s)  LowerLimitTransitionRegionWidth=0.1  LowerLimitTransitionRegionWidthUnits=deg  UpperLimitSpecify=off  UpperLimitBound=90  UpperLimitBoundUnits=deg  UpperLimitStiffness=1e4  UpperLimitStiffnessUnits=N*m/deg  UpperLimitDamping=10  UpperLimitDampingUnits=N*m/(deg/s)  UpperLimitTransitionRegionWidth=0.1  UpperLimitTransitionRegionWidthUnits=deg  TorqueActuationMode=NoTorque  MotionActuationMode=ComputedMotion  SensePosition=off  SenseVelocity=off  SenseAcceleration=off  SenseTorqueForce=off  SenseLowerLimitTorqueForce=off  SenseUpperLimitTorqueForce=off
  Transform Align Axis B : Suspension_Utilities/Transform Align Axis Three Points  pt1=hp_bcr_pivot.*rhs_hp  pt2=hp_pushrod_in.*rhs_hp  pt3=hp_bcr_shock  popup_f_axis=+Z
      settings: SourceProductName=SmCar - Suspension Utilites
  Transform Align Axis F : Suspension_Utilities/Transform Align Axis Three Points  pt1=hp_bcr_pivot.*rhs_hp  pt2=hp_pushrod_in.*rhs_hp  pt3=hp_bcr_shock  popup_f_axis=+Z
      settings: SourceProductName=SmCar - Suspension Utilites
  F : PMIOPort  Side=Right
  B : PMIOPort  Port=2  Side=Left
  connections:
  Transform Align Axis B/LConn1 -- B/RConn1
  Transform Align Axis F/RConn1 -- Revolute Bellcrank Pivot/RConn1
  Revolute Bellcrank Pivot/LConn1 -- Transform Align Axis B/RConn1
  Transform Align Axis F/LConn1 -- F/RConn1
